simulink model "lab_4_cont"  (R2024b)
settings: Solver=VariableStepAuto  StartTime=0.0  StopTime=0.3  RelTol=1e-3
values from neighbouring files (symbols this model uses):
  A = [-Ra/La -K/La; K/J 0]    [lab.m]
  Ad = expm(A*h)    [lab.m]
  B = [1/La  0; 0 -1/J]    [lab.m]
  Bd = double(int( expm(A*t) *  B, t, 0, h))    [lab.m]
  C = [1 0; 0 1]    [lab.m]
  Cd = C    [lab.m]
  D = [0 0; 0 0]    [lab.m]
  Dd = D    [lab.m]
  h = 0.01    [lab.m]
undefined symbols (not defined in the file or in its folder): den12z, den1z, den22z, den2z, num12z, num1z, num22z, num2z
settings Model: Creator=rober  LastModifiedBy=rober

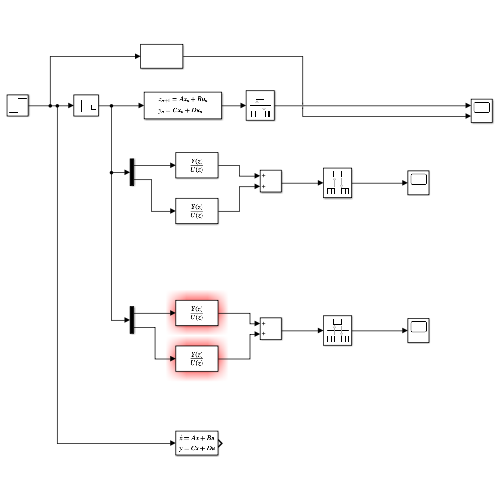
[thumbnail: Simulink's stored preview of the top-level diagram]
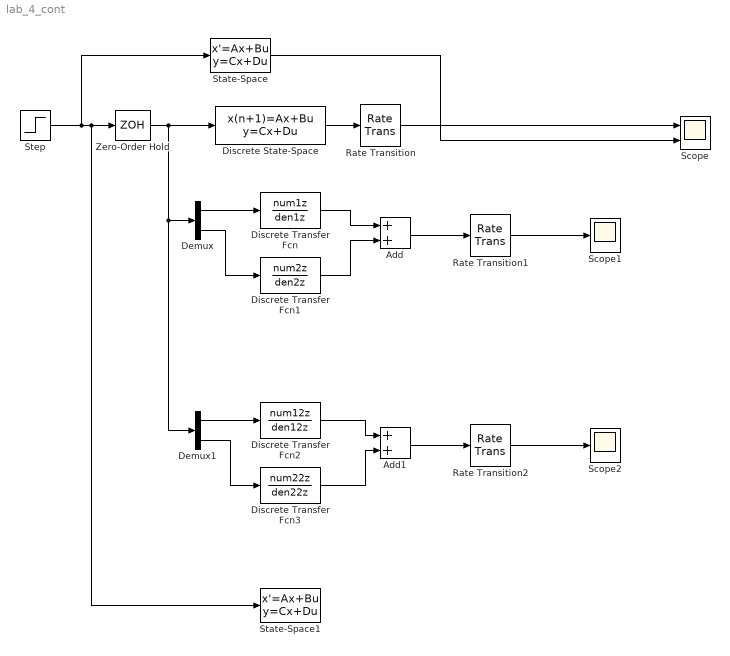
== system lab_4_cont ==
  Add : Sum
  Add1 : Sum
  Demux : Demux  Outputs=2
  Demux1 : Demux  Outputs=2
  Discrete Transfer Fcn : DiscreteTransferFcn  Numerator=num1z  Denominator=den1z
  Discrete Transfer Fcn1 : DiscreteTransferFcn  Numerator=num2z  Denominator=den2z
  Discrete Transfer Fcn2 : DiscreteTransferFcn  Numerator=num12z  Denominator=den12z
  Discrete Transfer Fcn3 : DiscreteTransferFcn  Numerator=num22z  Denominator=den22z
  Discrete State-Space : DiscreteStateSpace  A=Ad  B=Bd  C=Cd  D=Dd  SampleTime=h
  Rate Transition : RateTransition
  Rate Transition1 : RateTransition
  Rate Transition2 : RateTransition
  Scope : Scope  NumInputPorts=2
  Scope1 : Scope
  Scope2 : Scope
  State-Space : StateSpace  A=A  B=B  C=C  D=D  InitialCondition=0
  State-Space1 : StateSpace  A=A  B=B  C=C  D=D  InitialCondition=0
  Step : Step  Time=0  Before=[0, 0]  After=[24; 0.04]  SampleTime=h
  Zero-Order Hold : ZeroOrderHold  SampleTime=h
  wires:
  Step/1 -> State-Space/1, State-Space1/1, Zero-Order Hold/1
  Rate Transition/1 -> Scope/1
  Discrete State-Space/1 -> Rate Transition/1
  Demux/1 -> Discrete Transfer Fcn/1
  Demux/2 -> Discrete Transfer Fcn1/1
  Discrete Transfer Fcn/1 -> Add/1
  Discrete Transfer Fcn1/1 -> Add/2
  State-Space/1 -> Scope/2
  Add/1 -> Rate Transition1/1
  Rate Transition1/1 -> Scope1/1
  Zero-Order Hold/1 -> Demux1/1, Demux/1, Discrete State-Space/1
  Rate Transition2/1 -> Scope2/1
  Discrete Transfer Fcn3/1 -> Add1/2
  Add1/1 -> Rate Transition2/1
  Discrete Transfer Fcn2/1 -> Add1/1
  Demux1/1 -> Discrete Transfer Fcn2/1
  Demux1/2 -> Discrete Transfer Fcn3/1
